simulink model "dd"  (R2018b)
settings: Solver=VariableStepAuto  StartTime=0.0  StopTime=10.0  RelTol=1e-3
libraries: simulink x7
settings Model: Creator=Negar Pajooh  LastModifiedBy=Negar Pajooh

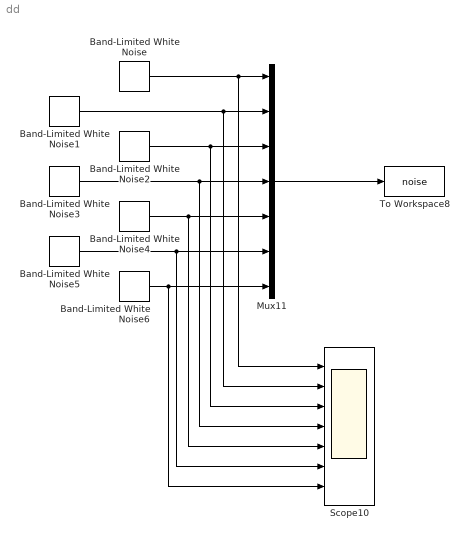
== system dd ==
  Band-Limited White Noise{,1..6} (7 alike) : simulink/Sources/Band-Limited White Noise  Cov=[0.1]  Ts=0.1  seed=[23341]
  Mux11 : Mux  Inputs=7
  Scope10 : Scope  NumInputPorts=7
  To Workspace8 : ToWorkspace  VariableName=noise  SampleTime=-1
      settings: Save2DSignal=2-D array (concatenate along first dimension)
  wires:
  Band-Limited White Noise2/1 -> Scope10/3, Mux11/3
  Band-Limited White Noise1/1 -> Scope10/2, Mux11/2
  Band-Limited White Noise/1 -> Scope10/1, Mux11/1
  Band-Limited White Noise4/1 -> Scope10/5, Mux11/5
  Band-Limited White Noise6/1 -> Scope10/7, Mux11/7
  Mux11/1 -> To Workspace8/1
  Band-Limited White Noise5/1 -> Scope10/6, Mux11/6
  Band-Limited White Noise3/1 -> Scope10/4, Mux11/4
